simulink model "torque_control"  (R2025b)
settings: Solver=FixedStepAuto  StartTime=0.0  StopTime=10.0  FixedStep=0.001  RelTol=1e-3
libraries: slpidlib x3, aerolibutil x2, matrix_library x1
settings Model: Creator=lew11  LastModifiedBy=rosette-nebula
settings DataIOCC: SaveFormat=StructureWithTime
settings OptimizationCC: BlockReduction=off  OptimizeBlockIOStorage=off  BufferReuse=off

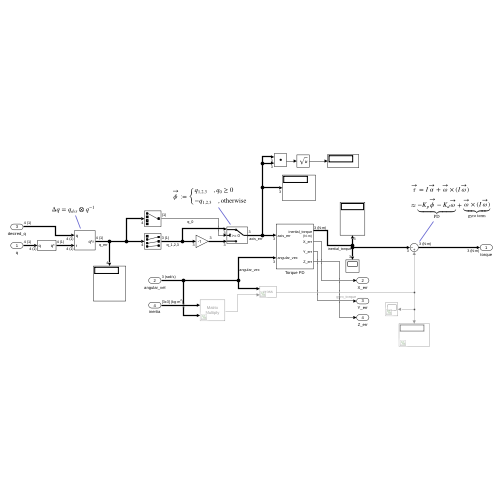
[thumbnail: Simulink's stored preview of the top-level diagram]
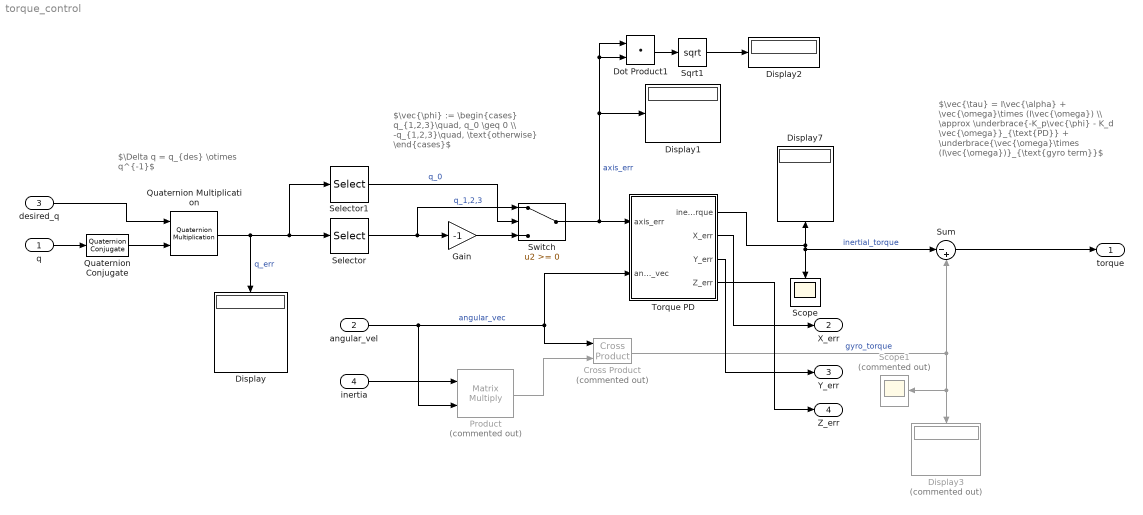
== system torque_control ==
  note: $\vec{\tau} = I\vec{\alpha} + \vec{\omega}\times (I\vec{\omega}) \\ \approx \underbrace{-K_p\vec{\phi} - K_d \vec{\omega}}_{\text{PD}} + \underbrace{\vec{\omega}\times (I\vec{\omega})}_{\text{gyro term}}$
  note: $\Delta q = q_{des} \otimes q^{-1}$
  note: $\vec{\phi} := \begin{cases} q_{1,2,3}\quad, q_0 \geq 0 \\ -q_{1,2,3}\quad, \text{otherwise} \end{cases}$
  q : Inport  PortDimensions=4
  angular_vel : Inport  Port=2  Unit=rad/s  PortDimensions=3
  desired_q : Inport  Port=3  PortDimensions=4
  inertia : Inport  Port=4  Unit=kg*m^2  PortDimensions=[3 3]
  Cross Product : matrix_library/Cross Product  Commented=on
  Display{,1..2,7} (4 alike) : Display
  Display3 : Display  Commented=on
  Dot Product1 : DotProduct  OutDataTypeStr=Inherit: Inherit via internal rule
  Gain : Gain  Gain=-1
  Product : Product  Commented=on  Multiplication=Matrix(*)
  Quaternion Conjugate : aerolibutil/Quaternion Conjugate
  Quaternion Multiplication : aerolibutil/Quaternion Multiplication
  Scope : Scope
      settings: ActiveDisplayYMinimum=-0.14932397347297444  ActiveDisplayYMaximum=0.07239216107669641
  Scope1 : Scope  Commented=on
      settings: ActiveDisplayYMinimum=0.0011947391550070411  ActiveDisplayYMaximum=0.0022299145437023543  DataLoggingVariableName=ScopeData2
  Selector : Selector  InputPortWidth=4  IndexOptions=Index vector (dialog)  Indices=[2 3 4]  OutputSizes=1
  Selector1 : Selector  InputPortWidth=4  IndexOptions=Index vector (dialog)  Indices=1  OutputSizes=1
  Sqrt1 : Sqrt  OutputSignalType=complex
  Sum : Sum  Inputs=|-+
  Switch : Switch  SaturateOnIntegerOverflow=off  InputSameDT=off
  Torque PD : Subsystem
  torque : Outport  Unit=N*m  PortDimensions=3
  X_err : Outport  Port=2
  Y_err : Outport  Port=3
  Z_err : Outport  Port=4
  wires:
  desired_q/1 -> Quaternion Multiplication/1
  q/1 -> Quaternion Conjugate/1
  Quaternion Conjugate/1 -> Quaternion Multiplication/2
  Quaternion Multiplication/1 -> Selector/1, Selector1/1, Display/1  "q_err"
  Selector1/1 -> Switch/2  "q_0"
  Selector/1 -> Gain/1, Switch/1  "q_1,2,3"
  Gain/1 -> Switch/3
  inertia/1 -> Product/1
  angular_vel/1 -> Cross Product/1, Torque PD/2(angular_vec), Product/2  "angular_vec"
  Sum/1 -> torque/1
  Cross Product/1 -> Display3/1, Scope1/1, Sum/2  "gyro_torque"
  Switch/1 -> Dot Product1/1, Dot Product1/2, Display1/1, Torque PD/1(axis_err)  "axis_err"
  Torque PD/1(inertial_torque) -> Sum/1, Scope/1, Display7/1  "inertial_torque"
  Dot Product1/1 -> Sqrt1/1
  Sqrt1/1 -> Display2/1
  Product/1 -> Cross Product/2
  Torque PD/2(X_err) -> X_err/1
  Torque PD/3(Y_err) -> Y_err/1
  Torque PD/4(Z_err) -> Z_err/1

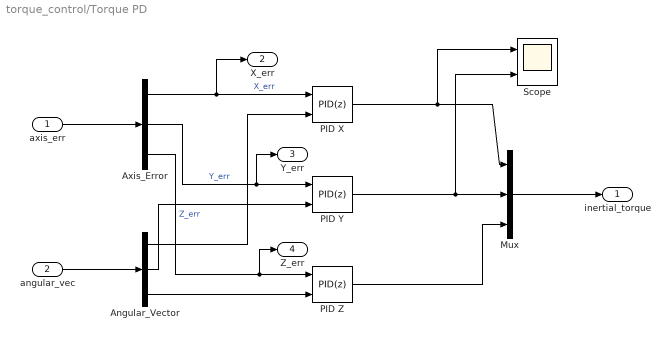
== system torque_control/Torque PD ==
  axis_err : Inport
  angular_vec : Inport  Port=2
  Angular_Vector : Demux  Outputs=3
  Axis_Error : Demux  Outputs=3
  Mux : Mux  Inputs=3
  PID X : slpidlib/PID Controller  Controller=PID  Form=Parallel  TimeDomain=Discrete-time  UseExternalTs=off  SampleTime=-1  IntegratorMethod=Forward Euler  FilterMethod=Forward Euler  ControllerParametersSource=internal  P=0  I=0.94146  UseKiTs=off  D=0  UseExternalDerivativeSource=on  N=100  UseFilter=off  TunerSelectOption=Transfer Function Based (PID Tuner App)  InitialConditionSource=internal  InitialConditionForIntegrator=0  InitialConditionForFilter=0  DifferentiatorICPrevScaledInput=0  ExternalReset=none  TrackingMode=off  Kt=1  LimitOutput=off  SatLimitsSource=internal  UpperSaturationLimit=inf  LowerSaturationLimit=-inf  LinearizeAsGain=on  AntiWindupMode=none  Kb=1  LimitIntegrator=off  UpperIntegratorSaturationLimit=inf  LowerIntegratorSaturationLimit=-inf  POutMin=[]  POutMax=[]  IOutMin=[]  IOutMax=[]  DOutMin=[]  DOutMax=[]  NOutMin=[]  NOutMax=[]  SumOutMin=[]  SumOutMax=[]  SaturationOutMin=[]  SaturationOutMax=[]  PParamMin=[]  PParamMax=[]  IParamMin=[]  IParamMax=[]  DParamMin=[]  DParamMax=[]  NParamMin=[]  NParamMax=[]  KbParamMin=[]  KbParamMax=[]  KtParamMin=[]  KtParamMax=[]  KbOutMin=[]  KbOutMax=[]  KtOutMin=[]  KtOutMax=[]  IntegratorOutMin=[]  IntegratorOutMax=[]  FilterOutMin=[]  FilterOutMax=[]  SumI1OutMin=[]  SumI1OutMax=[]  SumI2OutMin=[]  SumI2OutMax=[]  SumI3OutMin=[]  SumI3OutMax=[]  SumI4OutMin=[]  SumI4OutMax=[]  SumDOutMin=[]  SumDOutMax=[]  DifferentiatorOutMin=[]  DifferentiatorOutMax=[]  FilterDiffOutCoefMin=[]  FilterDiffOutCoefMax=[]  ReciprocalOutMin=[]  ReciprocalOutMax=[]  SumDenOutMin=[]  SumDenOutMax=[]  SumNumOutMin=[]  SumNumOutMax=[]  DivideOutMin=[]  DivideOutMax=[]  UdiffTsProdOutMin=[]  UdiffTsProdOutMax=[]  NTsProdOutMin=[]  NTsProdOutMax=[]  UintegralTsProdOutMin=[]  UintegralTsProdOutMax=[]  UngainTsProdOutMin=[]  UngainTsProdOutMax=[]  ClampingZeroOutDataTypeStr=Inherit: Inherit via back propagation  ClampingZeroOutMin=[]  ClampingZeroOutMax=[]  FilterDenConstantOutDataTypeStr=Inherit: Inherit via back propagation  FilterDenConstantOutMin=[]  FilterDenConstantOutMax=[]  PCopyOutDataTypeStr=Inherit: Inherit via back propagation  PCopyOutMin=[]  PCopyOutMax=[]  NCopyOutDataTypeStr=Inherit: Inherit via back propagation  NCopyOutMin=[]  NCopyOutMax=[]  IntegratorContinuousStateAttributes=''  IntegratorStateMustResolveToSignalObject=off  IntegratorRTWStateStorageClass=Auto  FilterContinuousStateAttributes=''  FilterStateMustResolveToSignalObject=off  FilterRTWStateStorageClass=Auto  ParallelPVariant=InternalParameters  IdealPVariant=Disabled  IVariant=InternalParameters  DVariant=InternalParameters  IntegratorVariant=Discrete  SatVariant=Disabled  AWVariant=Passthrough  PCopyVariant=Disabled  TRVariant=Disabled  FdbkBlocksVariant=Forward  IdealPFdbkVariant=Disabled  SatFdbkVariant=Disabled  DerivativeFilterVariant=Passthrough  NVariant=Passthrough  NCopyVariant=Disabled_SignalSpec  FilterICVariant=Disabled  IntegratorICVariant=InternalICs  ExternalResetVariant=Disabled  TRSumVariant=Passthrough  SumFdbkVariant=Disabled  SumVariant=Sum_PID  TsampFilterVariant=InternalTs  TsampNgainVariant=Passthrough  TsampIntegralVariant=Disabled_SignalSpec  ExternalSaturationOutDataTypeStr=Inherit: Same as second input  DerivativeSourceVariant=ExternalYdot  PreIntVariant=InternalPreInt
  PID Y : slpidlib/PID Controller  Controller=PID  Form=Parallel  TimeDomain=Discrete-time  UseExternalTs=off  SampleTime=-1  IntegratorMethod=Forward Euler  FilterMethod=Forward Euler  ControllerParametersSource=internal  P=2.3719  I=2.177  UseKiTs=off  D=0  UseExternalDerivativeSource=on  N=100  UseFilter=off  TunerSelectOption=Transfer Function Based (PID Tuner App)  InitialConditionSource=internal  InitialConditionForIntegrator=0  InitialConditionForFilter=0  DifferentiatorICPrevScaledInput=0  ExternalReset=none  TrackingMode=off  Kt=1  LimitOutput=off  SatLimitsSource=internal  UpperSaturationLimit=inf  LowerSaturationLimit=-inf  LinearizeAsGain=on  AntiWindupMode=none  Kb=1  LimitIntegrator=off  UpperIntegratorSaturationLimit=inf  LowerIntegratorSaturationLimit=-inf  POutMin=[]  POutMax=[]  IOutMin=[]  IOutMax=[]  DOutMin=[]  DOutMax=[]  NOutMin=[]  NOutMax=[]  SumOutMin=[]  SumOutMax=[]  SaturationOutMin=[]  SaturationOutMax=[]  PParamMin=[]  PParamMax=[]  IParamMin=[]  IParamMax=[]  DParamMin=[]  DParamMax=[]  NParamMin=[]  NParamMax=[]  KbParamMin=[]  KbParamMax=[]  KtParamMin=[]  KtParamMax=[]  KbOutMin=[]  KbOutMax=[]  KtOutMin=[]  KtOutMax=[]  IntegratorOutMin=[]  IntegratorOutMax=[]  FilterOutMin=[]  FilterOutMax=[]  SumI1OutMin=[]  SumI1OutMax=[]  SumI2OutMin=[]  SumI2OutMax=[]  SumI3OutMin=[]  SumI3OutMax=[]  SumI4OutMin=[]  SumI4OutMax=[]  SumDOutMin=[]  SumDOutMax=[]  DifferentiatorOutMin=[]  DifferentiatorOutMax=[]  FilterDiffOutCoefMin=[]  FilterDiffOutCoefMax=[]  ReciprocalOutMin=[]  ReciprocalOutMax=[]  SumDenOutMin=[]  SumDenOutMax=[]  SumNumOutMin=[]  SumNumOutMax=[]  DivideOutMin=[]  DivideOutMax=[]  UdiffTsProdOutMin=[]  UdiffTsProdOutMax=[]  NTsProdOutMin=[]  NTsProdOutMax=[]  UintegralTsProdOutMin=[]  UintegralTsProdOutMax=[]  UngainTsProdOutMin=[]  UngainTsProdOutMax=[]  ClampingZeroOutDataTypeStr=Inherit: Inherit via back propagation  ClampingZeroOutMin=[]  ClampingZeroOutMax=[]  FilterDenConstantOutDataTypeStr=Inherit: Inherit via back propagation  FilterDenConstantOutMin=[]  FilterDenConstantOutMax=[]  PCopyOutDataTypeStr=Inherit: Inherit via back propagation  PCopyOutMin=[]  PCopyOutMax=[]  NCopyOutDataTypeStr=Inherit: Inherit via back propagation  NCopyOutMin=[]  NCopyOutMax=[]  IntegratorContinuousStateAttributes=''  IntegratorStateMustResolveToSignalObject=off  IntegratorRTWStateStorageClass=Auto  FilterContinuousStateAttributes=''  FilterStateMustResolveToSignalObject=off  FilterRTWStateStorageClass=Auto  ParallelPVariant=InternalParameters  IdealPVariant=Disabled  IVariant=InternalParameters  DVariant=InternalParameters  IntegratorVariant=Discrete  SatVariant=Disabled  AWVariant=Passthrough  PCopyVariant=Disabled  TRVariant=Disabled  FdbkBlocksVariant=Forward  IdealPFdbkVariant=Disabled  SatFdbkVariant=Disabled  DerivativeFilterVariant=Passthrough  NVariant=Passthrough  NCopyVariant=Disabled_SignalSpec  FilterICVariant=Disabled  IntegratorICVariant=InternalICs  ExternalResetVariant=Disabled  TRSumVariant=Passthrough  SumFdbkVariant=Disabled  SumVariant=Sum_PID  TsampFilterVariant=InternalTs  TsampNgainVariant=Passthrough  TsampIntegralVariant=Disabled_SignalSpec  ExternalSaturationOutDataTypeStr=Inherit: Same as second input  DerivativeSourceVariant=ExternalYdot  PreIntVariant=InternalPreInt
  PID Z : slpidlib/PID Controller  Controller=PID  Form=Parallel  TimeDomain=Discrete-time  UseExternalTs=off  SampleTime=-1  IntegratorMethod=Forward Euler  FilterMethod=Forward Euler  ControllerParametersSource=internal  P=3.3627  I=3.1839  UseKiTs=off  D=5  UseExternalDerivativeSource=on  N=100  UseFilter=off  TunerSelectOption=Transfer Function Based (PID Tuner App)  InitialConditionSource=internal  InitialConditionForIntegrator=0  InitialConditionForFilter=0  DifferentiatorICPrevScaledInput=0  ExternalReset=none  TrackingMode=off  Kt=1  LimitOutput=off  SatLimitsSource=internal  UpperSaturationLimit=inf  LowerSaturationLimit=-inf  LinearizeAsGain=on  AntiWindupMode=none  Kb=1  LimitIntegrator=off  UpperIntegratorSaturationLimit=inf  LowerIntegratorSaturationLimit=-inf  POutMin=[]  POutMax=[]  IOutMin=[]  IOutMax=[]  DOutMin=[]  DOutMax=[]  NOutMin=[]  NOutMax=[]  SumOutMin=[]  SumOutMax=[]  SaturationOutMin=[]  SaturationOutMax=[]  PParamMin=[]  PParamMax=[]  IParamMin=[]  IParamMax=[]  DParamMin=[]  DParamMax=[]  NParamMin=[]  NParamMax=[]  KbParamMin=[]  KbParamMax=[]  KtParamMin=[]  KtParamMax=[]  KbOutMin=[]  KbOutMax=[]  KtOutMin=[]  KtOutMax=[]  IntegratorOutMin=[]  IntegratorOutMax=[]  FilterOutMin=[]  FilterOutMax=[]  SumI1OutMin=[]  SumI1OutMax=[]  SumI2OutMin=[]  SumI2OutMax=[]  SumI3OutMin=[]  SumI3OutMax=[]  SumI4OutMin=[]  SumI4OutMax=[]  SumDOutMin=[]  SumDOutMax=[]  DifferentiatorOutMin=[]  DifferentiatorOutMax=[]  FilterDiffOutCoefMin=[]  FilterDiffOutCoefMax=[]  ReciprocalOutMin=[]  ReciprocalOutMax=[]  SumDenOutMin=[]  SumDenOutMax=[]  SumNumOutMin=[]  SumNumOutMax=[]  DivideOutMin=[]  DivideOutMax=[]  UdiffTsProdOutMin=[]  UdiffTsProdOutMax=[]  NTsProdOutMin=[]  NTsProdOutMax=[]  UintegralTsProdOutMin=[]  UintegralTsProdOutMax=[]  UngainTsProdOutMin=[]  UngainTsProdOutMax=[]  ClampingZeroOutDataTypeStr=Inherit: Inherit via back propagation  ClampingZeroOutMin=[]  ClampingZeroOutMax=[]  FilterDenConstantOutDataTypeStr=Inherit: Inherit via back propagation  FilterDenConstantOutMin=[]  FilterDenConstantOutMax=[]  PCopyOutDataTypeStr=Inherit: Inherit via back propagation  PCopyOutMin=[]  PCopyOutMax=[]  NCopyOutDataTypeStr=Inherit: Inherit via back propagation  NCopyOutMin=[]  NCopyOutMax=[]  IntegratorContinuousStateAttributes=''  IntegratorStateMustResolveToSignalObject=off  IntegratorRTWStateStorageClass=Auto  FilterContinuousStateAttributes=''  FilterStateMustResolveToSignalObject=off  FilterRTWStateStorageClass=Auto  ParallelPVariant=InternalParameters  IdealPVariant=Disabled  IVariant=InternalParameters  DVariant=InternalParameters  IntegratorVariant=Discrete  SatVariant=Disabled  AWVariant=Passthrough  PCopyVariant=Disabled  TRVariant=Disabled  FdbkBlocksVariant=Forward  IdealPFdbkVariant=Disabled  SatFdbkVariant=Disabled  DerivativeFilterVariant=Passthrough  NVariant=Passthrough  NCopyVariant=Disabled_SignalSpec  FilterICVariant=Disabled  IntegratorICVariant=InternalICs  ExternalResetVariant=Disabled  TRSumVariant=Passthrough  SumFdbkVariant=Disabled  SumVariant=Sum_PID  TsampFilterVariant=InternalTs  TsampNgainVariant=Passthrough  TsampIntegralVariant=Disabled_SignalSpec  ExternalSaturationOutDataTypeStr=Inherit: Same as second input  DerivativeSourceVariant=ExternalYdot  PreIntVariant=InternalPreInt
  Scope : Scope  NumInputPorts=2
      settings: ActiveDisplayYMinimum=-0.051146207440445846  ActiveDisplayYMaximum=0.051198361947262412
  inertial_torque : Outport  Unit=N*m  PortDimensions=3
  X_err : Outport  Port=2
  Y_err : Outport  Port=3
  Z_err : Outport  Port=4
  wires:
  axis_err/1 -> Axis_Error/1
  Axis_Error/1 -> X_err/1, PID X/1  "X_err"
  Angular_Vector/3 -> PID Z/2
  Angular_Vector/1 -> PID X/2
  Angular_Vector/2 -> PID Y/2
  Axis_Error/3 -> Z_err/1, PID Z/1  "Z_err"
  Axis_Error/2 -> Y_err/1, PID Y/1  "Y_err"
  PID Y/1 -> Scope/2, Mux/2
  angular_vec/1 -> Angular_Vector/1
  PID Z/1 -> Mux/3
  PID X/1 -> Mux/1, Scope/1
  Mux/1 -> inertial_torque/1
